simulink model "sf_cycle_error_fix"  (R2025b)
settings: Solver=ode45  StartTime=0.0  StopTime=10.0  RelTol=1e-3  EnableMultiTasking=on
settings Model: FPTRunName=Active  ExtModeTrigMode=oneshot  ExtModeArmWhenConnect=off  ExtModeAutoUpdateStatusClock=off  Creator=The MathWorks, Inc.  LastModifiedBy=The MathWorks, Inc.
settings SolverCC: AlgebraicLoopSolver=TrustRegion  MaxZcPerStep=1.0
settings DataIOCC: SaveFormat=Array  ReturnWorkspaceOutputs=off
settings OptimizationCC: BooleanDataType=off  ReuseModelBlockBuffer=off  ExpressionDepthLimit=2147483647.0  InitFltsAndDblsToZero=on  LifeSpan=inf
settings DebuggingCC: SaveWithParameterizedLinksMsg=none  UnderspecifiedInitializationDetection=Classic  MergeDetectMultiDrivingBlocksExec=none  SignalResolutionControl=TryResolveAllWithWarning  MultiTaskDSMMsg=warning  MultiTaskCondExecSysMsg=none  FcnCallInpInsideContextMsg=warning  UnconnectedInputMsg=warning  UnconnectedOutputMsg=warning  UnconnectedLineMsg=warning  StateNameClashWarn=warning  SFUnexpectedBacktrackingDiag=warning  SFNoUnconditionalDefaultTransitionDiag=warning  SFExecutionAtInitializationDiag=none  ArithmeticOperatorsInVariantConditions=warning
settings HardwareCC: ProdBitPerPointer=32.0  ProdBitPerSizeT=32.0  ProdBitPerPtrDiffT=32.0  ProdLargestAtomicFloat=None  ProdIntDivRoundTo=Undefined  ProdEndianess=Unspecified  ProdWordSize=32.0  ProdHWDeviceType=32-bit Generic  TargetUnknown=on
settings ModelReferenceCC: EnableRefExpFcnMdlSchedulingChecks=on  PropagateSignalLabelsOutOfModel=off
settings SFSimCC: SimUseLocalCustomCode=off  SimParseCustomCode=off  CustomCodeUndefinedFunction=UseInterfaceOnly
settings RTWCC: RTWUseLocalCustomCode=off  GPUComputeCapability=3.5  DLArmComputeVersion=19.05
settings CodeAppCC: StateflowObjectComments=on
settings GRTTargetCC: TargetFcnLib=ansi_tfl_tmw.mat  TargetLangStandard=C89/C90 (ANSI)  CombineOutputUpdateFcns=off  GRTInterface=on
settings ConfigComp: CovMetricSettings=dcmtr  CovSaveCumulativeToWorkspaceVar=on  CovSaveSingleToWorkspaceVar=on  CovExternalEMLEnable=off  CovSFcnEnable=off

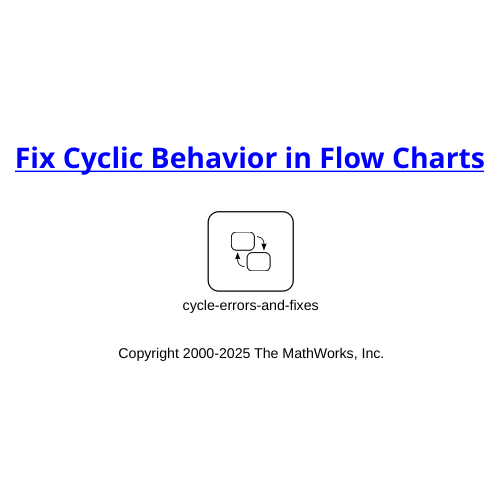
[thumbnail: Simulink's stored preview of the top-level diagram]
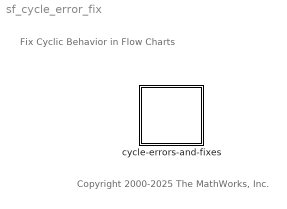
== system sf_cycle_error_fix ==
  note: Copyright 2000-2025 The MathWorks, Inc.
  note: Fix Cyclic Behavior in Flow Charts
  cycle-errors-and-fixes : Stateflow chart  TreatAsAtomicUnit=on

== stateflow chart sf_cycle_error_fix/cycle-errors-and-fixes ==
  state Error1 [function]
    note: The junctions in this loop
        | do not have an unconditional
        | path to a terminal junction.
    (default) -> (junction 23)
    (junction 24) -> (junction 23) [order 2] : [c2]
    (junction 23) -> (junction 24) : {action1;}
    (junction 24) -> (junction 25) [order 1] : [c1]
  state Fix1 [function]
    note: Incorporate the negation of condition c1
        | into the transition containing c2 so the
        | resulting diagram has an unconditional
        | path out of the loop.
    (default) -> (junction 26)
    (junction 27) -> (junction 26) [order 1] : [~c1 && c2]
    (junction 26) -> (junction 27) : {action1;}
    (junction 27) -> (junction 28) [order 2]
  state Error2 [function]
    note: The top junction in the loop
        | does not have an unconditional
        | path to a terminal junction.
    (default) -> (junction 56)
    (junction 60) -> (junction 56) [order 1] : [c2]
    (junction 56) -> (junction 60) : [c1]{action1;}
    (junction 60) -> (junction 53) [order 2] : {action2;}
  state Fix2 [function]
    note: Create an unconditional transition from
        | the top junction to the terminal junction.
    (default) -> (junction 32)
    (junction 32) -> (junction 34) [order 2]
    (junction 33) -> (junction 32) [order 1] : [c2]
    (junction 32) -> (junction 33) [order 1] : [c1]{action1;}
    (junction 33) -> (junction 34) [order 2] : {action2;}
  data: action1 local; action2 local; c1 local; c2 local
